simulink model "afe_rst_ctrl"  (R2026b)
settings: Solver=ode23t  StopTime=param.sim.simlength  FixedStep=tc  MaxStep=param.glb_time.tc  RelTol=1e-4
values from neighbouring files (symbols this model uses):
  param = add_template_extras(param, options)    [init_model.m]
undefined symbols (not defined in the file or in its folder): magnitude
libraries: fl_lib x181, nesl_utility x97, igbt_simple_2th_lib x6, afe_uvw_ctrl x5, discrete_time_low_pass_filter x2, threephase_inductor_lib x1, dclink_for_two_levels x1, three_phase_pwm_modulator x1, three_phase_inverter_ideal_switch_based_model x1, three_phase_inverter_mosfet_based_with_thermal_model x1, ee_lib x1, three_phase_voltage_with_frt_emulator_mfcn x1
(part 3 of 6)

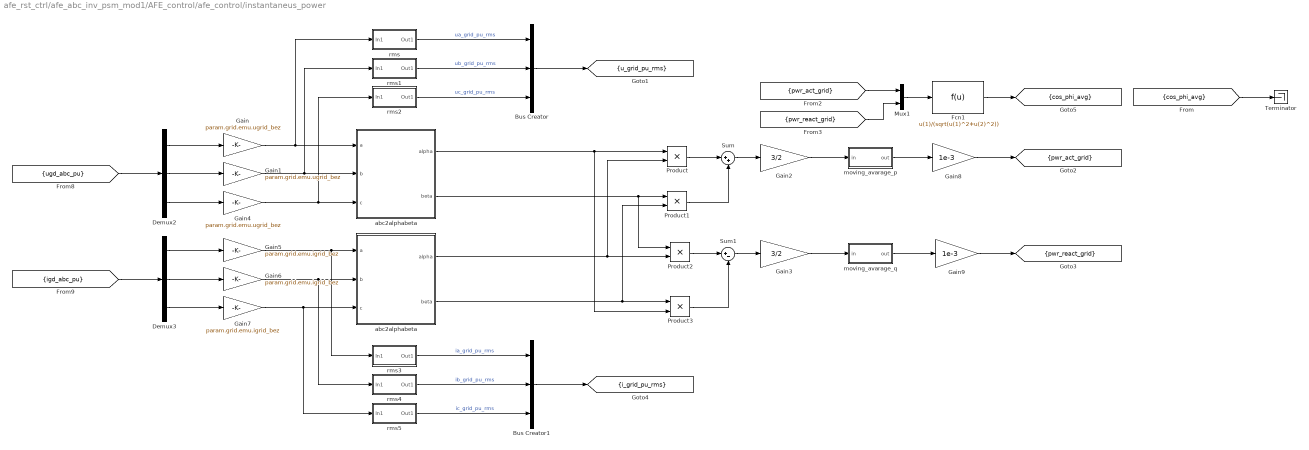
== system afe_rst_ctrl/afe_abc_inv_psm_mod1/AFE_control/afe_control/instantaneus_power ==
  Bus Creator : BusCreator  Inputs=3
  Bus Creator1 : BusCreator  Inputs=3
  Demux2 : Demux  Outputs=3
  Demux3 : Demux  Outputs=3
  Fcn1 : Fcn  Expr=u(1)/(sqrt(u(1)^2+u(2)^2))
  Gain : Gain  Gain=param.grid.emu.ugrid_bez
  Gain1 : Gain  Gain=param.grid.emu.ugrid_bez
  Gain2 : Gain  Gain=3/2
  Gain3 : Gain  Gain=3/2
  Gain4 : Gain  Gain=param.grid.emu.ugrid_bez
  Gain5 : Gain  Gain=param.grid.emu.igrid_bez
  Gain6 : Gain  Gain=param.grid.emu.igrid_bez
  Gain7 : Gain  Gain=param.grid.emu.igrid_bez
  Gain8 : Gain  Gain=1e-3
  Gain9 : Gain  Gain=1e-3
  Mux1 : Mux  Inputs=2
  Product{,1..3} (4 alike) : Product  RndMeth=Zero
  Sum : Sum  Inputs=|++
  Sum1 : Sum  Inputs=|+-
  Terminator : Terminator
  abc2alphabeta : Subsystem
  "abc2alphabeta " : Subsystem
  moving_avarage_p : Subsystem
  moving_avarage_q : Subsystem
  rms : Subsystem
  rms1 : Subsystem
  rms2 : Subsystem
  rms3 : Subsystem
  rms4 : Subsystem
  rms5 : Subsystem
  tag scope: cos_phi_avg=scoped, i_grid_pu_rms=scoped, pwr_act_grid=scoped, pwr_react_grid=scoped, u_grid_pu_rms=scoped
  wires:
  abc2alphabeta/2("beta ") -> Product1/1, Product2/1
  "abc2alphabeta "/2("beta ") -> Product1/2, Product3/1
  abc2alphabeta/1("alpha ") -> Product3/2, Product/1
  "abc2alphabeta "/1("alpha ") -> Product2/2, Product/2
  Product/1 -> Sum/1
  Product1/1 -> Sum/2
  Product2/1 -> Sum1/1
  Product3/1 -> Sum1/2
  Sum1/1 -> Gain3/1
  Sum/1 -> Gain2/1
  Gain2/1 -> moving_avarage_p/1(in)
  Gain3/1 -> moving_avarage_q/1(in)
  [pwr_react_grid] -> Mux1/2
  Mux1/1 -> Fcn1/1
  Fcn1/1 -> [cos_phi_avg]
  [pwr_act_grid] -> Mux1/1
  rms/1(Out1) -> Bus Creator/1  "ua_grid_pu_rms"
  rms2/1(Out1) -> Bus Creator/3  "uc_grid_pu_rms"
  rms1/1(Out1) -> Bus Creator/2  "ub_grid_pu_rms"
  moving_avarage_p/1(out) -> Gain8/1
  moving_avarage_q/1(out) -> Gain9/1
  Demux2/1 -> Gain/1
  Demux2/2 -> Gain1/1
  Demux2/3 -> Gain4/1
  Demux3/1 -> Gain5/1
  Demux3/2 -> Gain6/1
  Demux3/3 -> Gain7/1
  Gain/1 -> rms/1(In1), abc2alphabeta/1(a)
  Gain1/1 -> rms1/1(In1), abc2alphabeta/2(b)
  Gain4/1 -> rms2/1(In1), abc2alphabeta/3(c)
  Gain5/1 -> rms3/1(In1), "abc2alphabeta "/1(a)
  Gain6/1 -> rms4/1(In1), "abc2alphabeta "/2(b)
  Gain7/1 -> rms5/1(In1), "abc2alphabeta "/3(c)
  Gain8/1 -> [pwr_act_grid]
  Gain9/1 -> [pwr_react_grid]
  [ugd_abc_pu] -> Demux2/1
  [igd_abc_pu] -> Demux3/1
  Bus Creator/1 -> [u_grid_pu_rms]
  rms4/1(Out1) -> Bus Creator1/2  "ib_grid_pu_rms"
  rms3/1(Out1) -> Bus Creator1/1  "ia_grid_pu_rms"
  rms5/1(Out1) -> Bus Creator1/3  "ic_grid_pu_rms"
  Bus Creator1/1 -> [i_grid_pu_rms]
  [cos_phi_avg] -> Terminator/1

== system afe_rst_ctrl/afe_abc_inv_psm_mod1/AFE_control/afe_control/interesting scopes ==
  current_sequences_mod1 : Scope  NumInputPorts=4
      settings: ActiveDisplayYMinimum=-0.97178065031766891  ActiveDisplayYMaximum=1.9392475411295891  DataLoggingVariableName=ScopeData2
  i_grid_seq_ref : Scope
      settings: ActiveDisplayYMinimum=-1.1499999999999995  ActiveDisplayYMaximum=0.34999999999999981
  voltage_sequences_mod1 : Scope  NumInputPorts=4
      settings: ActiveDisplayYMinimum=-1.2405151816982258  ActiveDisplayYMaximum=1.2605257614333911
  wires:
  [v_grid_neg_eta_avg] -> voltage_sequences_mod1/4  "u_grid_neg_eta"
  [i_grid_neg_xi_avg] -> current_sequences_mod1/3  "i_grid_neg_xi"
  [v_grid_pos_eta_avg] -> voltage_sequences_mod1/2  "u_grid_pos_eta"
  [v_grid_neg_xi_avg] -> voltage_sequences_mod1/3  "u_grid_neg_xi"
  [i_grid_pos_xi_avg] -> current_sequences_mod1/1  "i_grid_pos_xi"
  [i_grid_neg_eta_avg] -> current_sequences_mod1/4  "i_grid_neg_eta"
  [v_grid_pos_xi_avg] -> voltage_sequences_mod1/1  "u_grid_pos_xi"
  [i_grid_pos_eta_avg] -> current_sequences_mod1/2  "i_grid_pos_eta"
  [i_grid_seq_ref] -> i_grid_seq_ref/1  "i_grid_seq_ref"

== system afe_rst_ctrl/afe_abc_inv_psm_mod1/AFE_control/afe_control/is afe quantizzation and one step delay ==
  is_abc_pu : Inport
  Demux : Demux  Outputs=3
  Mux : Mux  Inputs=3
  is afe quantizzation and one step delay : Subsystem
  isd_abc_pu : Outport
  wires:
  is afe quantizzation and one step delay/2(isd_v_pu) -> Mux/2
  is_abc_pu/1 -> Demux/1
  is afe quantizzation and one step delay/3(isd_w_pu) -> Mux/3
  is afe quantizzation and one step delay/1(isd_u_pu) -> Mux/1
  Demux/1 -> is afe quantizzation and one step delay/1(is_u_pu)
  Mux/1 -> isd_abc_pu/1
  Demux/3 -> is afe quantizzation and one step delay/3(is_w_pu)
  Demux/2 -> is afe quantizzation and one step delay/2(is_v_pu)

== system afe_rst_ctrl/afe_abc_inv_psm_mod1/AFE_control/afe_control/islanding_mode_detector ==
  gamma : Inport
  alpha : Inport  Port=2
  beta : Inport  Port=3
  Constant : Constant
  Mux : Mux  Inputs=2
  island_detection : Scope  NumInputPorts=3
      settings: ActiveDisplayYMinimum=-13.028939727220205  ActiveDisplayYMaximum=117.26045754498188  DataLoggingVariableName=ScopeData10
  islanding_detector : afe_uvw_ctrl/islanding_detector  p=param.afe.uvw
  wires:
  Mux/1 -> islanding_detector/1
  alpha/1 -> Mux/1  "u_grid_alpha"
  beta/1 -> Mux/2  "u_grid_beta"
  gamma/1 -> islanding_detector/2  "gamma_grid"
  [omega_grid_pll_pu] -> islanding_detector/3
  Constant/1 -> islanding_detector/4
  islanding_detector/1 -> island_detection/1
  islanding_detector/2 -> island_detection/2
  islanding_detector/3 -> island_detection/3

== system afe_rst_ctrl/afe_abc_inv_psm_mod1/AFE_control/afe_control/phase_compensation_1 ==
  local_time : Inport
  master_time : Inport  Port=2
  Zero-Order Hold : ZeroOrderHold  SampleTime=-1
  Zero-Order Hold1 : ZeroOrderHold  SampleTime=-1
  alignment_eval_afe1 : Subsystem
  y : Outport
  wires:
  local_time/1 -> Zero-Order Hold/1
  master_time/1 -> Zero-Order Hold1/1
  alignment_eval_afe1/1(dp) -> y/1
  Zero-Order Hold/1 -> alignment_eval_afe1/1(local_time)
  Zero-Order Hold1/1 -> alignment_eval_afe1/2(master_time)

== system afe_rst_ctrl/afe_abc_inv_psm_mod1/AFE_control/afe_control/space_vector ==
  uab_out : Inport
  Bus Creator : BusCreator  Inputs=3
  Bus Selector : BusSelector  OutputSignals=da,db,dc
  C Caller : CCaller  FunctionName=sv_pwm_cm_process_simulink  PortSpecificationStruct="%)30     .    B H   8    (     @         %    \"     8    !     0         %  0 \"0    $    _    07)G3F%M90  4&]R=$YA;64 4V-O<&4     26YD97@     5'EP90      4VEZ90      27-';&]B86P   X    P    !@    @    $          4    (     0    ,    !         !   P!O=70 #@   #     &    \"     0         !0    @    !     P    $         $  # &]U=  .    .     8    (    !          %    \"     $    &     0         0   ...(+3252 chars)"
  Constant : Constant  Value=param.glb_time.ts_afe
  Constant1 : Constant
  Data Type Conversion1 : DataTypeConversion  OutDataTypeStr=double  SaturateOnIntegerOverflow=off  RndMeth=Floor
  Data Type Conversion{4,15..16,18} (4 alike) : DataTypeConversion  OutDataTypeStr=single  SaturateOnIntegerOverflow=off  RndMeth=Floor
  Data Type Conversion17 : DataTypeConversion  OutDataTypeStr=uint32  SaturateOnIntegerOverflow=off  RndMeth=Floor
  Data Type Conversion2 : DataTypeConversion  OutDataTypeStr=double  SaturateOnIntegerOverflow=off  RndMeth=Floor
  Data Type Conversion3 : DataTypeConversion  OutDataTypeStr=double  SaturateOnIntegerOverflow=off  RndMeth=Floor
  Demux : Demux  Outputs=3
  Gain1 : Gain  Gain=sqrt(3)/2
  Gain2 : Gain  Gain=sqrt(3)/2
  Gain3 : Gain  Gain=param.afe.ref.u_cm_comp_mod1
  duvw : Outport
  wires:
  Data Type Conversion15/1 -> C Caller/2
  Bus Selector/2 -> Data Type Conversion2/1  "<db>"
  Data Type Conversion18/1 -> C Caller/1
  C Caller/1 -> Bus Selector/1
  Bus Creator/1 -> duvw/1
  Data Type Conversion1/1 -> Bus Creator/1  "du(k)"
  Demux/2 -> Gain2/1
  Bus Selector/3 -> Data Type Conversion3/1  "<dc>"
  Demux/1 -> Gain1/1
  Data Type Conversion2/1 -> Bus Creator/2  "dv(k)"
  Gain2/1 -> Data Type Conversion15/1
  Bus Selector/1 -> Data Type Conversion1/1  "<da>"
  Gain1/1 -> Data Type Conversion18/1
  Data Type Conversion3/1 -> Bus Creator/3  "dw(k)"
  Constant/1 -> Data Type Conversion16/1
  uab_out/1 -> Demux/1
  Constant1/1 -> Data Type Conversion17/1
  Data Type Conversion16/1 -> C Caller/4
  Data Type Conversion17/1 -> C Caller/5
  Demux/3 -> Gain3/1
  Gain3/1 -> Data Type Conversion4/1
  Data Type Conversion4/1 -> C Caller/3

== system afe_rst_ctrl/afe_abc_inv_psm_mod1/AFE_control/afe_control/udc_acquisition ==
  udc_pu : Inport
  Quantizer : Quantizer  QuantizationInterval=param.meas.adc_quantization
  Unit Delay : UnitDelay  SampleTime=-1
  Zero-Order Hold : ZeroOrderHold  SampleTime=-1
  udcd_pu : Outport
  wires:
  Quantizer/1 -> Unit Delay/1
  udc_pu/1 -> Zero-Order Hold/1
  Unit Delay/1 -> udcd_pu/1
  Zero-Order Hold/1 -> Quantizer/1

== system afe_rst_ctrl/afe_abc_inv_psm_mod1/AFE_control/afe_control/udc_ctrl ==
  udc_pu : Inport
  1/Ti : Gain  Gain=param.afe.ctrl.kp_udc_ctrl  SaturateOnIntegerOverflow=on  OutDataTypeStr=Inherit: Same as input  ParamDataTypeStr=Inherit: Same as input
  Constant : Constant  Value=0
  Gain : Gain  Gain=-1
  Saturation : Saturate  UpperLimit=param.afe.ctrl.ixi_pos_ref_lim  LowerLimit=-param.afe.ctrl.ixi_pos_ref_lim
  Sum1 : Sum  Inputs=+++  SaturateOnIntegerOverflow=on
  Sum2 : Sum  Inputs=-+  SaturateOnIntegerOverflow=on
  Sum3 : Sum  Inputs=-+  SaturateOnIntegerOverflow=on
  Switch : Switch  Criteria=u2 > Threshold  SaturateOnIntegerOverflow=off  InputSameDT=off
  To Workspace1 : ToWorkspace  VariableName=udc_pu_sim_mod1  SampleTime=-1
      settings: MaxDataPoints=param.glb_time.Ns_afe
  To Workspace3 : ToWorkspace  VariableName=udc_pu_ref_sim_mod1  SampleTime=-1
      settings: MaxDataPoints=param.glb_time.Ns_afe
  Unit Delay4 : UnitDelay  SampleTime=-1
  discrete-time-low-pass-filter1 : discrete_time_low_pass_filter/discrete-time-low-pass-filter  tau=20e-3  ts=param.glb_time.ts_afe
  kp : Gain  Gain=param.afe.ctrl.ki_udc_ctrl*param.glb_time.ts_afe  SaturateOnIntegerOverflow=on  OutDataTypeStr=Inherit: Same as input  ParamDataTypeStr=Inherit: Same as input
  udc_norm_ref : Step  Time=1e-3  FinalValue=param.afe.ctrl.udc_norm_ref
  udc_tracking : Scope  NumInputPorts=3
      settings: ActiveDisplayYMinimum=-2.0004150390624997  ActiveDisplayYMaximum=1.5037353515624998  DataLoggingVariableName=ScopeData8
  i_xi_ref : Outport
  wires:
  1/Ti/1 -> Sum1/1, Sum3/1
  kp/1 -> Sum1/2
  Sum3/1 -> Unit Delay4/1
  Unit Delay4/1 -> Sum1/3
  udc_norm_ref/1 -> discrete-time-low-pass-filter1/1
  udc_pu/1 -> Sum2/1, To Workspace1/1, udc_tracking/2  "udc_pu"
  Sum2/1 -> kp/1, 1/Ti/1
  Sum1/1 -> Saturation/1
  [pwr_lim_enable] -> Switch/2
  Saturation/1 -> Switch/3
  Switch/1 -> Sum3/2, Gain/1
  Constant/1 -> Switch/1
  Gain/1 -> udc_tracking/3, i_xi_ref/1  "i_xi_ref"
  discrete-time-low-pass-filter1/1 -> To Workspace3/1, udc_tracking/1, Sum2/2  "udc_pu_ref"

== system afe_rst_ctrl/afe_abc_inv_psm_mod1/AFE_control/afe_control/ug afe quantizzation and one step delay ==
  ug_abc_pu : Inport
  Demux : Demux  Outputs=3
  Mux : Mux  Inputs=3
  ug afe quantizzation and one step delay : Subsystem
  ugd_abc_pu : Outport
  wires:
  ug afe quantizzation and one step delay/2(ugd_v_pu) -> Mux/2
  Demux/2 -> ug afe quantizzation and one step delay/2(ug_v_pu)
  Demux/3 -> ug afe quantizzation and one step delay/3(ug_w_pu)
  ug afe quantizzation and one step delay/1(ugd_u_pu) -> Mux/1
  Demux/1 -> ug afe quantizzation and one step delay/1(ug_u_pu)
  ug_abc_pu/1 -> Demux/1
  ug afe quantizzation and one step delay/3(ugd_w_pu) -> Mux/3
  Mux/1 -> ugd_abc_pu/1

== system afe_rst_ctrl/afe_abc_inv_psm_mod1/afe/sv_pwm/modulator1 ==
  u : Inport
  v : Inport  Port=2
  w : Inport  Port=3
  phase : Inport  Port=4
  Bus Creator : BusCreator  Inputs=3
  Three phase two level PWM generator with global TRGO : three_phase_pwm_modulator/Three phase two level PWM generator with global TRGO  f=param.glb_time.fPWM_AFE  m_up=0.98  m_low=0.02  dead_time=param.glb_time.dead_time_AFE  pos_cmd_gate=15  neg_cmd_gate=-10  polarity=1  tc=param.glb_time.tc  double_sampling=1
      link override gate commands/Bus Selector: OutputSignals=du(t)
      link override gate commands/Bus Selector1: OutputSignals=dv(t)
      link override gate commands/Bus Selector2: OutputSignals=dw(t)
  gate_cmds : Outport
  tag scope: TRGO_afe_module_1=global
  wires:
  [time_afe_module_1] -> Three phase two level PWM generator with global TRGO/1
  Bus Creator/1 -> Three phase two level PWM generator with global TRGO/3
  Three phase two level PWM generator with global TRGO/1 -> [TRGO_afe_module_1]
  u/1 -> Bus Creator/1
  v/1 -> Bus Creator/2
  w/1 -> Bus Creator/3
  phase/1 -> Three phase two level PWM generator with global TRGO/2
  Three phase two level PWM generator with global TRGO/2 -> gate_cmds/1

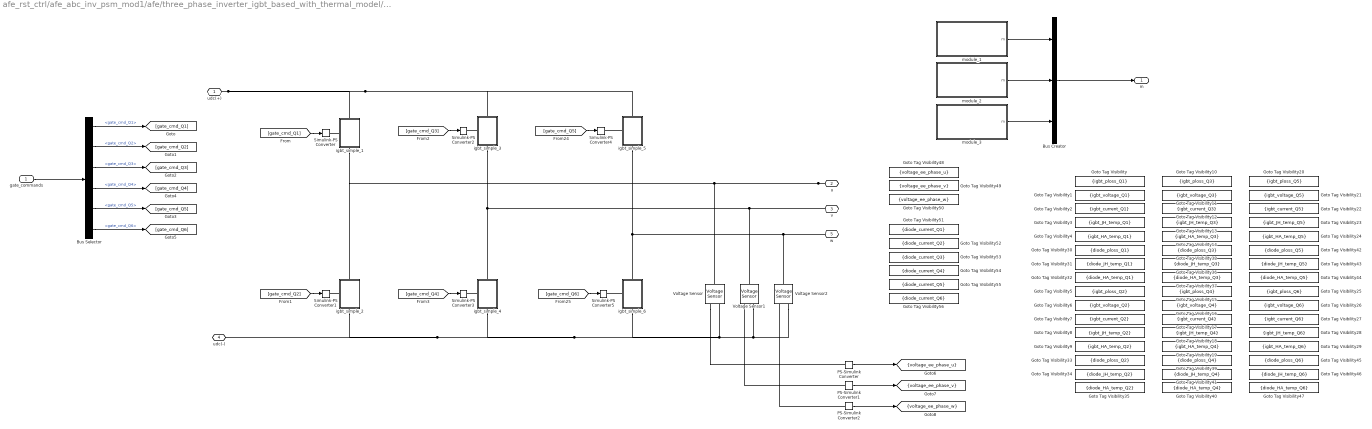
== system afe_rst_ctrl/afe_abc_inv_psm_mod1/afe/three_phase_inverter_igbt_based_with_thermal_model/three_phase_inverter_with_igbt_simple_2th ==
  gate_commands : Inport
  Bus Creator : BusCreator  Inputs=3
  Bus Selector : BusSelector  OutputSignals=gate_cmd_Q1,gate_cmd_Q2,gate_cmd_Q3,gate_cmd_Q4,gate_cmd_Q5,gate_cmd_Q6
  Goto Tag Visibility : GotoTagVisibility  GotoTag=igbt_ploss_Q1
  Goto Tag Visibility1 : GotoTagVisibility  GotoTag=igbt_voltage_Q1
  Goto Tag Visibility10 : GotoTagVisibility  GotoTag=igbt_ploss_Q3
  Goto Tag Visibility11 : GotoTagVisibility  GotoTag=igbt_voltage_Q3
  Goto Tag Visibility12 : GotoTagVisibility  GotoTag=igbt_current_Q3
  Goto Tag Visibility13 : GotoTagVisibility  GotoTag=igbt_JH_temp_Q3
  Goto Tag Visibility14 : GotoTagVisibility  GotoTag=igbt_HA_temp_Q3
  Goto Tag Visibility15 : GotoTagVisibility  GotoTag=igbt_ploss_Q4
  Goto Tag Visibility16 : GotoTagVisibility  GotoTag=igbt_voltage_Q4
  Goto Tag Visibility17 : GotoTagVisibility  GotoTag=igbt_current_Q4
  Goto Tag Visibility18 : GotoTagVisibility  GotoTag=igbt_JH_temp_Q4
  Goto Tag Visibility19 : GotoTagVisibility  GotoTag=igbt_HA_temp_Q4
  Goto Tag Visibility2 : GotoTagVisibility  GotoTag=igbt_current_Q1
  Goto Tag Visibility20 : GotoTagVisibility  GotoTag=igbt_ploss_Q5
  Goto Tag Visibility21 : GotoTagVisibility  GotoTag=igbt_voltage_Q5
  Goto Tag Visibility22 : GotoTagVisibility  GotoTag=igbt_current_Q5
  Goto Tag Visibility23 : GotoTagVisibility  GotoTag=igbt_JH_temp_Q5
  Goto Tag Visibility24 : GotoTagVisibility  GotoTag=igbt_HA_temp_Q5
  Goto Tag Visibility25 : GotoTagVisibility  GotoTag=igbt_ploss_Q6
  Goto Tag Visibility26 : GotoTagVisibility  GotoTag=igbt_voltage_Q6
  Goto Tag Visibility27 : GotoTagVisibility  GotoTag=igbt_current_Q6
  Goto Tag Visibility28 : GotoTagVisibility  GotoTag=igbt_JH_temp_Q6
  Goto Tag Visibility29 : GotoTagVisibility  GotoTag=igbt_HA_temp_Q6
  Goto Tag Visibility3 : GotoTagVisibility  GotoTag=igbt_JH_temp_Q1
  Goto Tag Visibility30 : GotoTagVisibility  GotoTag=diode_ploss_Q1
  Goto Tag Visibility31 : GotoTagVisibility  GotoTag=diode_JH_temp_Q1
  Goto Tag Visibility32 : GotoTagVisibility  GotoTag=diode_HA_temp_Q1
  Goto Tag Visibility33 : GotoTagVisibility  GotoTag=diode_ploss_Q2
  Goto Tag Visibility34 : GotoTagVisibility  GotoTag=diode_JH_temp_Q2
  Goto Tag Visibility35 : GotoTagVisibility  GotoTag=diode_HA_temp_Q2
  Goto Tag Visibility36 : GotoTagVisibility  GotoTag=diode_JH_temp_Q3
  Goto Tag Visibility37 : GotoTagVisibility  GotoTag=diode_HA_temp_Q3
  Goto Tag Visibility38 : GotoTagVisibility  GotoTag=diode_ploss_Q3
  Goto Tag Visibility39 : GotoTagVisibility  GotoTag=diode_ploss_Q4
  Goto Tag Visibility4 : GotoTagVisibility  GotoTag=igbt_HA_temp_Q1
  Goto Tag Visibility40 : GotoTagVisibility  GotoTag=diode_HA_temp_Q4
  Goto Tag Visibility41 : GotoTagVisibility  GotoTag=diode_JH_temp_Q4
  Goto Tag Visibility42 : GotoTagVisibility  GotoTag=diode_ploss_Q5
  Goto Tag Visibility43 : GotoTagVisibility  GotoTag=diode_JH_temp_Q5
  Goto Tag Visibility44 : GotoTagVisibility  GotoTag=diode_HA_temp_Q5
  Goto Tag Visibility45 : GotoTagVisibility  GotoTag=diode_ploss_Q6
  Goto Tag Visibility46 : GotoTagVisibility  GotoTag=diode_JH_temp_Q6
  Goto Tag Visibility47 : GotoTagVisibility  GotoTag=diode_HA_temp_Q6
  Goto Tag Visibility48 : GotoTagVisibility  GotoTag=voltage_ee_phase_u
  Goto Tag Visibility49 : GotoTagVisibility  GotoTag=voltage_ee_phase_v
  Goto Tag Visibility5 : GotoTagVisibility  GotoTag=igbt_ploss_Q2
  Goto Tag Visibility50 : GotoTagVisibility  GotoTag=voltage_ee_phase_w
  Goto Tag Visibility51 : GotoTagVisibility  GotoTag=diode_current_Q1
  Goto Tag Visibility52 : GotoTagVisibility  GotoTag=diode_current_Q2
  Goto Tag Visibility53 : GotoTagVisibility  GotoTag=diode_current_Q3
  Goto Tag Visibility54 : GotoTagVisibility  GotoTag=diode_current_Q4
  Goto Tag Visibility55 : GotoTagVisibility  GotoTag=diode_current_Q5
  Goto Tag Visibility56 : GotoTagVisibility  GotoTag=diode_current_Q6
  Goto Tag Visibility6 : GotoTagVisibility  GotoTag=igbt_voltage_Q2
  Goto Tag Visibility7 : GotoTagVisibility  GotoTag=igbt_current_Q2
  Goto Tag Visibility8 : GotoTagVisibility  GotoTag=igbt_JH_temp_Q2
  Goto Tag Visibility9 : GotoTagVisibility  GotoTag=igbt_HA_temp_Q2
  PS-Simulink Converter : nesl_utility/PS-Simulink Converter  PhysicalDomain=network_engine_domain  SubClassName=ps_output  LeftPortType=input  RightPortType=output  PseudoPeriodic=off  Frequencies=[]  VectorFormat=1-D array  Unit=V  AffineConversion=off
  PS-Simulink Converter1 : nesl_utility/PS-Simulink Converter  PhysicalDomain=network_engine_domain  SubClassName=ps_output  LeftPortType=input  RightPortType=output  PseudoPeriodic=off  Frequencies=[]  VectorFormat=1-D array  Unit=V  AffineConversion=off
  PS-Simulink Converter2 : nesl_utility/PS-Simulink Converter  PhysicalDomain=network_engine_domain  SubClassName=ps_output  LeftPortType=input  RightPortType=output  PseudoPeriodic=off  Frequencies=[]  VectorFormat=1-D array  Unit=V  AffineConversion=off
  Simulink-PS Converter{,1..5} (6 alike) : nesl_utility/Simulink-PS Converter  PhysicalDomain=network_engine_domain  SubClassName=ps_input  LeftPortType=input  RightPortType=output  PseudoPeriodic=off  Frequencies=[]  NoiseDistribution=none  NoiseParameters=[]  Unit=V  AffineConversion=off  FilteringAndDerivatives=provide  SimscapeFilterOrder=1  InputFilterTimeConstant=0.001  UdotUserProvided=0
  Voltage Sensor : fl_lib/Electrical/Electrical Sensors/Voltage Sensor
  Voltage Sensor1 : fl_lib/Electrical/Electrical Sensors/Voltage Sensor
  Voltage Sensor2 : fl_lib/Electrical/Electrical Sensors/Voltage Sensor
  igbt_simple_1 : Subsystem
      settings: PortSchema="{\"entries\":[{\"content\":{\"sides\":[{\"content\":{\"connectorIds\":[\"LConn1\"]},\"type\":\"ConnectorPlacement.EquallySpacedRectSide\",\"uuid\":\"9277da8d-d460-43e6-8478-dd662f15d226\"},{\"content\":{\"connectorIds\":[],\"side\":\"RIGHT\"},\"type\":\"ConnectorPlacement.EquallySpacedRectSide\",\"uuid\":\"a7ece396-f1d9-4f4f-a05b-db1fc65d6e1d\"},{\"content\":{\"connectorIds\":[\"LConn2\"],\"side\":\"TOP\"},\"type\":\"ConnectorPlacement.EquallySpacedRectSide\",\"uuid\":\"fdd70777-e9cf-4317-afb6-cae87f75d5b0\"},{\"content\":{\"connectorIds\":[\"RConn1\"],\"side\":\"BOTTOM\"},\"type\":\"ConnectorPlacement.EquallySpacedRectSide\",\"uuid\":\"2353ed68-b1a1-4775-9ca9-31e268d5443b\"}]},\"type\":\"ConnectorPlacement.EquallySpacedConnector\",\"uuid\":\"d5479f4c-4e65-4791-adcb-73df11f88590\"}],\"packageUris\":[\"http://schema.mathworks.com/mf0/Connector/R2020b\"],\"version\":\"1.0\"}"
  igbt_simple_2 : Subsystem
      settings: PortSchema="{\"entries\":[{\"content\":{\"sides\":[{\"content\":{\"connectorIds\":[\"LConn1\"]},\"type\":\"ConnectorPlacement.EquallySpacedRectSide\",\"uuid\":\"9277da8d-d460-43e6-8478-dd662f15d226\"},{\"content\":{\"connectorIds\":[],\"side\":\"RIGHT\"},\"type\":\"ConnectorPlacement.EquallySpacedRectSide\",\"uuid\":\"a7ece396-f1d9-4f4f-a05b-db1fc65d6e1d\"},{\"content\":{\"connectorIds\":[\"LConn2\"],\"side\":\"TOP\"},\"type\":\"ConnectorPlacement.EquallySpacedRectSide\",\"uuid\":\"fdd70777-e9cf-4317-afb6-cae87f75d5b0\"},{\"content\":{\"connectorIds\":[\"RConn1\"],\"side\":\"BOTTOM\"},\"type\":\"ConnectorPlacement.EquallySpacedRectSide\",\"uuid\":\"2353ed68-b1a1-4775-9ca9-31e268d5443b\"}]},\"type\":\"ConnectorPlacement.EquallySpacedConnector\",\"uuid\":\"d5479f4c-4e65-4791-adcb-73df11f88590\"}],\"packageUris\":[\"http://schema.mathworks.com/mf0/Connector/R2020b\"],\"version\":\"1.0\"}"
  igbt_simple_3 : Subsystem
      settings: PortSchema="{\"entries\":[{\"content\":{\"sides\":[{\"content\":{\"connectorIds\":[\"LConn1\"]},\"type\":\"ConnectorPlacement.EquallySpacedRectSide\",\"uuid\":\"9277da8d-d460-43e6-8478-dd662f15d226\"},{\"content\":{\"connectorIds\":[],\"side\":\"RIGHT\"},\"type\":\"ConnectorPlacement.EquallySpacedRectSide\",\"uuid\":\"a7ece396-f1d9-4f4f-a05b-db1fc65d6e1d\"},{\"content\":{\"connectorIds\":[\"LConn2\"],\"side\":\"TOP\"},\"type\":\"ConnectorPlacement.EquallySpacedRectSide\",\"uuid\":\"fdd70777-e9cf-4317-afb6-cae87f75d5b0\"},{\"content\":{\"connectorIds\":[\"RConn1\"],\"side\":\"BOTTOM\"},\"type\":\"ConnectorPlacement.EquallySpacedRectSide\",\"uuid\":\"2353ed68-b1a1-4775-9ca9-31e268d5443b\"}]},\"type\":\"ConnectorPlacement.EquallySpacedConnector\",\"uuid\":\"d5479f4c-4e65-4791-adcb-73df11f88590\"}],\"packageUris\":[\"http://schema.mathworks.com/mf0/Connector/R2020b\"],\"version\":\"1.0\"}"
  igbt_simple_4 : Subsystem
      settings: PortSchema="{\"entries\":[{\"content\":{\"sides\":[{\"content\":{\"connectorIds\":[\"LConn1\"]},\"type\":\"ConnectorPlacement.EquallySpacedRectSide\",\"uuid\":\"9277da8d-d460-43e6-8478-dd662f15d226\"},{\"content\":{\"connectorIds\":[],\"side\":\"RIGHT\"},\"type\":\"ConnectorPlacement.EquallySpacedRectSide\",\"uuid\":\"a7ece396-f1d9-4f4f-a05b-db1fc65d6e1d\"},{\"content\":{\"connectorIds\":[\"LConn2\"],\"side\":\"TOP\"},\"type\":\"ConnectorPlacement.EquallySpacedRectSide\",\"uuid\":\"fdd70777-e9cf-4317-afb6-cae87f75d5b0\"},{\"content\":{\"connectorIds\":[\"RConn1\"],\"side\":\"BOTTOM\"},\"type\":\"ConnectorPlacement.EquallySpacedRectSide\",\"uuid\":\"2353ed68-b1a1-4775-9ca9-31e268d5443b\"}]},\"type\":\"ConnectorPlacement.EquallySpacedConnector\",\"uuid\":\"d5479f4c-4e65-4791-adcb-73df11f88590\"}],\"packageUris\":[\"http://schema.mathworks.com/mf0/Connector/R2020b\"],\"version\":\"1.0\"}"
  igbt_simple_5 : Subsystem
      settings: PortSchema="{\"entries\":[{\"content\":{\"sides\":[{\"content\":{\"connectorIds\":[\"LConn1\"]},\"type\":\"ConnectorPlacement.EquallySpacedRectSide\",\"uuid\":\"9277da8d-d460-43e6-8478-dd662f15d226\"},{\"content\":{\"connectorIds\":[],\"side\":\"RIGHT\"},\"type\":\"ConnectorPlacement.EquallySpacedRectSide\",\"uuid\":\"a7ece396-f1d9-4f4f-a05b-db1fc65d6e1d\"},{\"content\":{\"connectorIds\":[\"LConn2\"],\"side\":\"TOP\"},\"type\":\"ConnectorPlacement.EquallySpacedRectSide\",\"uuid\":\"fdd70777-e9cf-4317-afb6-cae87f75d5b0\"},{\"content\":{\"connectorIds\":[\"RConn1\"],\"side\":\"BOTTOM\"},\"type\":\"ConnectorPlacement.EquallySpacedRectSide\",\"uuid\":\"2353ed68-b1a1-4775-9ca9-31e268d5443b\"}]},\"type\":\"ConnectorPlacement.EquallySpacedConnector\",\"uuid\":\"d5479f4c-4e65-4791-adcb-73df11f88590\"}],\"packageUris\":[\"http://schema.mathworks.com/mf0/Connector/R2020b\"],\"version\":\"1.0\"}"
  igbt_simple_6 : Subsystem
      settings: PortSchema="{\"entries\":[{\"content\":{\"sides\":[{\"content\":{\"connectorIds\":[\"LConn1\"]},\"type\":\"ConnectorPlacement.EquallySpacedRectSide\",\"uuid\":\"9277da8d-d460-43e6-8478-dd662f15d226\"},{\"content\":{\"connectorIds\":[],\"side\":\"RIGHT\"},\"type\":\"ConnectorPlacement.EquallySpacedRectSide\",\"uuid\":\"a7ece396-f1d9-4f4f-a05b-db1fc65d6e1d\"},{\"content\":{\"connectorIds\":[\"LConn2\"],\"side\":\"TOP\"},\"type\":\"ConnectorPlacement.EquallySpacedRectSide\",\"uuid\":\"fdd70777-e9cf-4317-afb6-cae87f75d5b0\"},{\"content\":{\"connectorIds\":[\"RConn1\"],\"side\":\"BOTTOM\"},\"type\":\"ConnectorPlacement.EquallySpacedRectSide\",\"uuid\":\"2353ed68-b1a1-4775-9ca9-31e268d5443b\"}]},\"type\":\"ConnectorPlacement.EquallySpacedConnector\",\"uuid\":\"d5479f4c-4e65-4791-adcb-73df11f88590\"}],\"packageUris\":[\"http://schema.mathworks.com/mf0/Connector/R2020b\"],\"version\":\"1.0\"}"
  module_1 : Subsystem
  module_2 : Subsystem
  module_3 : Subsystem
  udc(+) : PMIOPort  Side=Left
  u : PMIOPort  Port=2  Side=Right
  v : PMIOPort  Port=3  Side=Right
  udc(-) : PMIOPort  Port=4  Side=Left
  w : PMIOPort  Port=5  Side=Right
  m : Outport
  tag scope: voltage_ee_phase_u=scoped, voltage_ee_phase_v=scoped, voltage_ee_phase_w=scoped
  wires:
  module_3/1(m) -> Bus Creator/3
  module_1/1(m) -> Bus Creator/1
  Bus Creator/1 -> m/1
  module_2/1(m) -> Bus Creator/2
  PS-Simulink Converter2/1 -> [voltage_ee_phase_w]
  PS-Simulink Converter1/1 -> [voltage_ee_phase_v]
  PS-Simulink Converter/1 -> [voltage_ee_phase_u]
  Bus Selector/6 -> [gate_cmd_Q6]  "<gate_cmd_Q6>"
  Bus Selector/5 -> [gate_cmd_Q5]  "<gate_cmd_Q5>"
  [gate_cmd_Q6] -> Simulink-PS Converter5/1
  [gate_cmd_Q5] -> Simulink-PS Converter4/1
  [gate_cmd_Q3] -> Simulink-PS Converter2/1
  Bus Selector/2 -> [gate_cmd_Q2]  "<gate_cmd_Q2>"
  Bus Selector/1 -> [gate_cmd_Q1]  "<gate_cmd_Q1>"
  Bus Selector/3 -> [gate_cmd_Q3]  "<gate_cmd_Q3>"
  [gate_cmd_Q4] -> Simulink-PS Converter3/1
  [gate_cmd_Q2] -> Simulink-PS Converter1/1
  [gate_cmd_Q1] -> Simulink-PS Converter/1
  Bus Selector/4 -> [gate_cmd_Q4]  "<gate_cmd_Q4>"
  gate_commands/1 -> Bus Selector/1
  connections:
  PS-Simulink Converter2/LConn1 -- Voltage Sensor2/RConn1
  PS-Simulink Converter1/LConn1 -- Voltage Sensor1/RConn1
  Voltage Sensor/RConn1 -- PS-Simulink Converter/LConn1
  w/RConn1 -- Voltage Sensor2/LConn1 -- igbt_simple_6/LConn2 -- igbt_simple_5/RConn1
  v/RConn1 -- Voltage Sensor1/LConn1 -- igbt_simple_4/LConn2 -- igbt_simple_3/RConn1
  Voltage Sensor1/RConn2 -- Voltage Sensor2/RConn2 -- Voltage Sensor/RConn2 -- igbt_simple_6/RConn1 -- igbt_simple_4/RConn1 -- igbt_simple_2/RConn1 -- udc(-)/RConn1
  igbt_simple_6/LConn1 -- Simulink-PS Converter5/RConn1
  igbt_simple_5/LConn1 -- Simulink-PS Converter4/RConn1
  igbt_simple_4/LConn1 -- Simulink-PS Converter3/RConn1
  igbt_simple_3/LConn1 -- Simulink-PS Converter2/RConn1
  igbt_simple_2/LConn1 -- Simulink-PS Converter1/RConn1
  igbt_simple_1/LConn1 -- Simulink-PS Converter/RConn1
  udc(+)/RConn1 -- igbt_simple_1/LConn2 -- igbt_simple_5/LConn2 -- igbt_simple_3/LConn2
  u/RConn1 -- Voltage Sensor/LConn1 -- igbt_simple_2/LConn2 -- igbt_simple_1/RConn1

== system afe_rst_ctrl/afe_abc_inv_psm_mod1/AFE_control/afe_control/FRT-VDE4110/positive_reactive_current_reference ==
  Step : Step  Time=param.afe.ref.time_i_react_pos_ref_1  InitialValue=param.afe.ref.i_react_pos_ref_1  FinalValue=param.afe.ref.i_react_pos_ref_2
  Step1 : Step  Time=param.afe.ref.time_i_react_pos_ref_2  FinalValue=param.afe.ref.i_react_pos_ref_3-param.afe.ref.i_react_pos_ref_2
  Sum7 : Sum  Inputs=|++
  i_react_pos_ref : Outport
  wires:
  Sum7/1 -> i_react_pos_ref/1
  Step1/1 -> Sum7/2
  Step/1 -> Sum7/1

== system afe_rst_ctrl/afe_abc_inv_psm_mod1/AFE_control/afe_control/current_ctrl1/current_transformation ==
  is_a_pu : Inport
  is_b_pu : Inport  Port=2
  is_c_pu : Inport  Port=3
  alphabeta2xieta : MATLAB Function  TreatAsAtomicUnit=on
  uvw2alphabeta : MATLAB Function  TreatAsAtomicUnit=on
  tag scope: id_eta_pu=scoped, id_xi_pu=scoped
  wires:
  is_c_pu/1 -> uvw2alphabeta/3(w)
  alphabeta2xieta/2(eta) -> [id_eta_pu]  "ieta_pu"
  alphabeta2xieta/1(xi) -> [id_xi_pu]  "ixi_pu"
  is_b_pu/1 -> uvw2alphabeta/2(v)
  uvw2alphabeta/2(beta) -> alphabeta2xieta/2(beta)  "ibeta_pu"
  uvw2alphabeta/1(alpha) -> alphabeta2xieta/1(alpha)  "ialpha_pu"
  [phase_grid_pll] -> alphabeta2xieta/3(gamma)
  is_a_pu/1 -> uvw2alphabeta/1(u)

== system afe_rst_ctrl/afe_abc_inv_psm_mod1/AFE_control/afe_control/current_ctrl1/inner_current_ctrl ==
  In1 : Inport
  is_abc : Inport  Port=2
  Mux : Mux  Inputs=3
  Selector : Selector  InputPortWidth=3  IndexOptions=Index vector (dialog)  Indices=[1]  OutputSizes=1  RuntimeRangeChecks=off
  Selector1 : Selector  InputPortWidth=3  IndexOptions=Index vector (dialog)  Indices=[1]  OutputSizes=1  RuntimeRangeChecks=off
  Selector2 : Selector  InputPortWidth=3  IndexOptions=Index vector (dialog)  Indices=[2]  OutputSizes=1  RuntimeRangeChecks=off
  Selector3 : Selector  InputPortWidth=3  IndexOptions=Index vector (dialog)  Indices=[2]  OutputSizes=1  RuntimeRangeChecks=off
  Selector4 : Selector  InputPortWidth=3  IndexOptions=Index vector (dialog)  Indices=[3]  OutputSizes=1  RuntimeRangeChecks=off
  Selector5 : Selector  InputPortWidth=3  IndexOptions=Index vector (dialog)  Indices=[3]  OutputSizes=1  RuntimeRangeChecks=off
  isa_ref/isa : Scope  NumInputPorts=2
      settings: ActiveDisplayYMinimum=0.46634443711045703  ActiveDisplayYMaximum=1.1209185909366344
  isb_ref/isb : Scope  NumInputPorts=2
      settings: ActiveDisplayYMinimum=-1.381866613392059  ActiveDisplayYMaximum=1.3822246036957448  DataLoggingVariableName=ScopeData2
  isc_ref/isc : Scope  NumInputPorts=2
      settings: ActiveDisplayYMinimum=-1.9270596811485752  ActiveDisplayYMaximum=1.9769102920110639  DataLoggingVariableName=ScopeData3
  rpi_phase_a : Subsystem
  rpi_phase_b : Subsystem
  rpi_phase_c : Subsystem
  zero_current_ctrl : Subsystem
  uabg : Outport  VectorParamsAs1DForOutWhenUnconnected=off
  tag scope: isa=scoped, isa_ref=scoped, isb=scoped, isb_ref=scoped, isc=scoped, isc_ref=scoped
  wires:
  In1/1 -> Selector4/1, Selector2/1, Selector/1  "isd_abc_pu_ref"
  is_abc/1 -> Selector5/1, Selector3/1, Selector1/1  "isd_abc_pu"
  Selector/1 -> [isa_ref], isa_ref/isa/1, rpi_phase_a/1(In1)  "isa_ref"
  Selector1/1 -> [isa], isa_ref/isa/2, rpi_phase_a/2(In2)  "isa"
  Selector2/1 -> rpi_phase_b/1(In1), [isb_ref], isb_ref/isb/1  "isb_ref"
  Selector3/1 -> rpi_phase_b/2(In2), [isb], isb_ref/isb/2  "isb"
  Selector4/1 -> rpi_phase_c/1(In1), [isc_ref], isc_ref/isc/1  "isc_ref"
  Selector5/1 -> rpi_phase_c/2(In2), [isc], isc_ref/isc/2  "isc"
  rpi_phase_a/1(Out1) -> Mux/1  "da"
  rpi_phase_b/1(Out1) -> Mux/2  "db"
  rpi_phase_c/1(Out1) -> Mux/3  "dc"
  Mux/1 -> zero_current_ctrl/1(d_abc)  "d_abc"
  zero_current_ctrl/1(u_ctrl_out) -> uabg/1

== system afe_rst_ctrl/afe_abc_inv_psm_mod1/AFE_control/afe_control/current_ctrl1/xieta2abc_ref ==
  pos_xi_ref : Inport
  pos_eta : Inport  Port=2
  neg_xi : Inport  Port=3
  neg_eta : Inport  Port=4
  phase : Inport  Port=5
  MATLAB Function2 : MATLAB Function  TreatAsAtomicUnit=on
  Mux : Mux  Inputs=3
  Negative Sequence : MATLAB Function  TreatAsAtomicUnit=on
  Positive Sequence : MATLAB Function  TreatAsAtomicUnit=on
  Sum : Sum  Inputs=|++
  Sum1 : Sum  Inputs=|++
  i_abc_ref : Outport
  wires:
  neg_eta/1 -> Negative Sequence/2(eta)
  MATLAB Function2/1(a) -> Mux/1  "i_a"
  Positive Sequence/2(beta) -> Sum1/1
  Sum/1 -> MATLAB Function2/1(alpha)
  phase/1 -> Negative Sequence/3(phase), Positive Sequence/3(phase)
  MATLAB Function2/3(c) -> Mux/3  "i_c"
  Negative Sequence/1(alpha) -> Sum/2
  Positive Sequence/1(alpha) -> Sum/1
  Negative Sequence/2(beta) -> Sum1/2
  MATLAB Function2/2(b) -> Mux/2  "i_b"
  Sum1/1 -> MATLAB Function2/2(beta)
  neg_xi/1 -> Negative Sequence/1(xi)
  pos_xi_ref/1 -> Positive Sequence/1(xi)
  pos_eta/1 -> Positive Sequence/2(eta)
  Mux/1 -> i_abc_ref/1  "i_abc"

== system afe_rst_ctrl/afe_abc_inv_psm_mod1/AFE_control/afe_control/data_to_worspace_module_1/dq_pll ==
  Bus Creator1 : BusCreator  Inputs=8
  dqPLLs : Outport
  wires:
  [phase_grid_fht_simulink_pll] -> Bus Creator1/5  "phase_grid_fht_simulink_pll"
  [omega_grid_fht_simulink_pll] -> Bus Creator1/6  "omega_grid_fht_simulink_pll"
  [omega_grid_fhtsr_dqpll] -> Bus Creator1/8  "omega_grid_fhtsr_dqpll"
  [phase_grid_fhtsr_dqpll] -> Bus Creator1/7  "phase_grid_fhtsr_dqpll"
  [omega_grid_dqpll_ccaller] -> Bus Creator1/4  "omega_grid_dqpll_ccaller"
  [phase_grid_dqpll_ccaller] -> Bus Creator1/3  "phase_grid_dqpll_ccaller"
  [omega_grid_pu_dqpll] -> Bus Creator1/2  "omega_grid_pu_dqpll"
  [phase_grid_dqpll] -> Bus Creator1/1  "phase_grid_dqpll"
  Bus Creator1/1 -> dqPLLs/1

== system afe_rst_ctrl/afe_abc_inv_psm_mod1/AFE_control/afe_control/data_to_worspace_module_1/inner_current_tracking ==
  Bus Creator1 : BusCreator  Inputs=11
  m_inner_current_tracking : Outport
  wires:
  [iz_pu] -> Bus Creator1/10  "iz_pu"
  [id_eta_pu] -> Bus Creator1/2  "i_eta_pu"
  [isc] -> Bus Creator1/8  "isc_pu"
  [isa_ref] -> Bus Creator1/3  "isa_pu_ref"
  [isa] -> Bus Creator1/4  "isa_pu"
  [id_xi_pu] -> Bus Creator1/1  "i_xi_pu"
  [iz_pu_ref] -> Bus Creator1/9  "iz_pu_ref"
  [isb] -> Bus Creator1/6  "isb_pu"
  [isb_ref] -> Bus Creator1/5  "isb_pu_ref"
  [iz_ctrl_out] -> Bus Creator1/11  "iz_ctrl_out"
  [isc_ref] -> Bus Creator1/7  "isc_pu_ref"
  Bus Creator1/1 -> m_inner_current_tracking/1

== system afe_rst_ctrl/afe_abc_inv_psm_mod1/AFE_control/afe_control/data_to_worspace_module_1/pwr_meter ==
  Bus Creator1 : BusCreator  Inputs=4
  m_pwr_meter : Outport
  wires:
  [u_grid_pu_rms] -> Bus Creator1/2  "u_grid_pu_rms"
  Bus Creator1/1 -> m_pwr_meter/1
  [pwr_act_grid] -> Bus Creator1/3  "pwr_act_grid"
  [pwr_react_grid] -> Bus Creator1/4  "pwr_react_grid"
  [i_grid_pu_rms] -> Bus Creator1/1  "i_grid_pu_rms"

== system afe_rst_ctrl/afe_abc_inv_psm_mod1/AFE_control/afe_control/data_to_worspace_module_1/sequences_data ==
  Bus Creator1 : BusCreator  Inputs=11
  Demux : Demux  Outputs=3
  m_seq : Outport
  wires:
  Bus Creator1/1 -> m_seq/1
  Demux/3 -> Bus Creator1/3  "i_grid_neg_eta_ref"
  Demux/2 -> Bus Creator1/2  "i_grid_neg_xi_ref"
  Demux/1 -> Bus Creator1/1  "i_grid_pos_eta_ref"
  [v_grid_pos_xi_avg] -> Bus Creator1/4  "v_grid_pos_xi_avg"
  [v_grid_pos_eta_avg] -> Bus Creator1/5  "v_grid_pos_eta_avg"
  [v_grid_neg_xi_avg] -> Bus Creator1/6  "v_grid_neg_xi_avg"
  [v_grid_neg_eta_avg] -> Bus Creator1/7  "v_grid_neg_eta_avg"
  [i_grid_pos_xi_avg] -> Bus Creator1/8  "i_grid_pos_xi_avg"
  [i_grid_pos_eta_avg] -> Bus Creator1/9  "i_grid_pos_eta_avg"
  [i_grid_neg_xi_avg] -> Bus Creator1/10  "i_grid_neg_xi_avg"
  [i_grid_neg_eta_avg] -> Bus Creator1/11  "i_grid_neg_eta_avg"
  [i_grid_seq_ref] -> Demux/1

== system afe_rst_ctrl/afe_abc_inv_psm_mod1/AFE_control/afe_control/grid_voltage_phase_lock_loops/FHT-PLL_simulink ==
  ug_abc_pu : Inport
  pll_stageA : Subsystem
  pll_stageB : Subsystem
  gamma_grid_fht_pll : Outport
  omega_grid_fht_pll : Outport  Port=2
  wires:
  pll_stageB/1(gamma_grid_ddsrf_pll) -> pll_stageA/1(gamma_grid), gamma_grid_fht_pll/1
  pll_stageA/2(u_grid_eta) -> pll_stageB/2(u_grid_pos_eta)  "u_grid_pos_eta"
  pll_stageA/1(u_grid_xi) -> pll_stageB/1(u_grid_pos_xi)  "u_grid_pos_xi"
  pll_stageB/2(omega_grid_ddsrf_pll) -> omega_grid_fht_pll/1
  ug_abc_pu/1 -> pll_stageA/2(ug_abc_pu)

== system afe_rst_ctrl/afe_abc_inv_psm_mod1/AFE_control/afe_control/ig afe quantizzation and one step delay/ig afe quantizzation and one step delay ==
  ig_u_pu : Inport
  ig_v_pu : Inport  Port=2
  ig_w_pu : Inport  Port=3
  Gain4 : Gain  Gain=-1
  Gain5 : Gain  Gain=-1
  Gain6 : Gain  Gain=-1
  Quantizer1 : Quantizer  QuantizationInterval=param.meas.adc_quantization
  Quantizer2 : Quantizer  QuantizationInterval=param.meas.adc_quantization
  Quantizer4 : Quantizer  QuantizationInterval=param.meas.adc_quantization
  Unit Delay : UnitDelay  SampleTime=-1
  Unit Delay1 : UnitDelay  SampleTime=-1
  Unit Delay2 : UnitDelay  SampleTime=-1
  Zero-Order Hold : ZeroOrderHold  SampleTime=-1
  Zero-Order Hold1 : ZeroOrderHold  SampleTime=-1
  Zero-Order Hold2 : ZeroOrderHold  SampleTime=-1
  igd_u_pu : Outport
  igd_v_pu : Outport  Port=2
  igd_w_pu : Outport  Port=3
  wires:
  Quantizer1/1 -> Unit Delay1/1
  Quantizer4/1 -> Unit Delay/1
  Quantizer2/1 -> Unit Delay2/1
  ig_u_pu/1 -> Zero-Order Hold/1
  ig_v_pu/1 -> Zero-Order Hold1/1
  ig_w_pu/1 -> Zero-Order Hold2/1
  Unit Delay/1 -> Gain4/1
  Unit Delay1/1 -> Gain5/1
  Unit Delay2/1 -> Gain6/1
  Gain4/1 -> igd_u_pu/1
  Gain5/1 -> igd_v_pu/1
  Gain6/1 -> igd_w_pu/1
  Zero-Order Hold/1 -> Quantizer4/1
  Zero-Order Hold1/1 -> Quantizer1/1
  Zero-Order Hold2/1 -> Quantizer2/1

== system afe_rst_ctrl/afe_abc_inv_psm_mod1/AFE_control/afe_control/instantaneus_power/abc2alphabeta ==
  a : Inport
  b : Inport  Port=2
  c : Inport  Port=3
  Gain1 : Gain  Gain=-1/2
  Gain11 : Gain  Gain=-1/2
  Gain2 : Gain  Gain=0
  Gain3 : Gain  Gain=sqrt(3)/2
  Gain4 : Gain  Gain=-sqrt(3)/2
  Gain8 : Gain  Gain=2/3
  Gain9 : Gain  Gain=2/3
  Sum : Sum  Inputs=+++
  Sum1 : Sum  Inputs=+++
  "alpha " : Outport  VectorParamsAs1DForOutWhenUnconnected=off
  "beta " : Outport  Port=2  VectorParamsAs1DForOutWhenUnconnected=off
  wires:
  Gain3/1 -> Sum1/2
  Gain2/1 -> Sum1/1
  Gain11/1 -> Sum/2
  Gain4/1 -> Sum1/3
  Sum1/1 -> Gain9/1
  Gain8/1 -> "alpha "/1
  Sum/1 -> Gain8/1
  c/1 -> Gain4/1, Gain1/1
  Gain9/1 -> "beta "/1
  b/1 -> Gain3/1, Gain11/1
  Gain1/1 -> Sum/3
  a/1 -> Gain2/1, Sum/1

== system afe_rst_ctrl/afe_abc_inv_psm_mod1/AFE_control/afe_control/instantaneus_power/abc2alphabeta  ==
  a : Inport
  b : Inport  Port=2
  c : Inport  Port=3
  Gain1 : Gain  Gain=-1/2
  Gain11 : Gain  Gain=-1/2
  Gain2 : Gain  Gain=0
  Gain3 : Gain  Gain=sqrt(3)/2
  Gain4 : Gain  Gain=-sqrt(3)/2
  Gain8 : Gain  Gain=2/3
  Gain9 : Gain  Gain=2/3
  Sum : Sum  Inputs=+++
  Sum1 : Sum  Inputs=+++
  "alpha " : Outport  VectorParamsAs1DForOutWhenUnconnected=off
  "beta " : Outport  Port=2  VectorParamsAs1DForOutWhenUnconnected=off
  wires:
  a/1 -> Sum/1, Gain2/1
  Gain2/1 -> Sum1/1
  Gain9/1 -> "beta "/1
  Gain11/1 -> Sum/2
  c/1 -> Gain1/1, Gain4/1
  Sum/1 -> Gain8/1
  Sum1/1 -> Gain9/1
  Gain1/1 -> Sum/3
  Gain3/1 -> Sum1/2
  Gain4/1 -> Sum1/3
  Gain8/1 -> "alpha "/1
  b/1 -> Gain11/1, Gain3/1

== system afe_rst_ctrl/afe_abc_inv_psm_mod1/AFE_control/afe_control/instantaneus_power/moving_avarage_p ==
  in : Inport
  Gain : Gain  Gain=param.afe.ctrl.rms.n1-1
  Gain1 : Gain  Gain=1/param.afe.ctrl.rms.n1
  Sum : Sum  Inputs=|++
  Unit Delay : UnitDelay  SampleTime=-1
  out : Outport  VectorParamsAs1DForOutWhenUnconnected=off
  wires:
  Gain/1 -> Sum/2
  Gain1/1 -> out/1, Unit Delay/1
  in/1 -> Sum/1
  Unit Delay/1 -> Gain/1
  Sum/1 -> Gain1/1

== system afe_rst_ctrl/afe_abc_inv_psm_mod1/AFE_control/afe_control/instantaneus_power/moving_avarage_q ==
  in : Inport
  Gain : Gain  Gain=param.afe.ctrl.rms.n1-1
  Gain1 : Gain  Gain=1/param.afe.ctrl.rms.n1
  Sum : Sum  Inputs=|++
  Unit Delay : UnitDelay  SampleTime=-1
  out : Outport  VectorParamsAs1DForOutWhenUnconnected=off
  wires:
  Sum/1 -> Gain1/1
  Unit Delay/1 -> Gain/1
  in/1 -> Sum/1
  Gain1/1 -> Unit Delay/1, out/1
  Gain/1 -> Sum/2

== system afe_rst_ctrl/afe_abc_inv_psm_mod1/AFE_control/afe_control/instantaneus_power/rms ==
  In1 : Inport
  Gain : Gain  Gain=param.afe.ctrl.rms.n10-1
  Gain1 : Gain  Gain=1/param.afe.ctrl.rms.n10
  Math Function : Math  Operator=magnitude^2  SignedPower=on
  Sqrt : Sqrt
  Sum : Sum  Inputs=|++
  Unit Delay : UnitDelay  SampleTime=-1
  Out1 : Outport  VectorParamsAs1DForOutWhenUnconnected=off
  wires:
  In1/1 -> Math Function/1
  Sum/1 -> Gain1/1
  Gain1/1 -> Sqrt/1, Unit Delay/1
  Unit Delay/1 -> Gain/1
  Math Function/1 -> Sum/1
  Sqrt/1 -> Out1/1
  Gain/1 -> Sum/2

== system afe_rst_ctrl/afe_abc_inv_psm_mod1/AFE_control/afe_control/instantaneus_power/rms1 ==
  In1 : Inport
  Gain : Gain  Gain=param.afe.ctrl.rms.n10-1
  Gain1 : Gain  Gain=1/param.afe.ctrl.rms.n10
  Math Function : Math  Operator=magnitude^2  SignedPower=on
  Sqrt : Sqrt
  Sum : Sum  Inputs=|++
  Unit Delay : UnitDelay  SampleTime=-1
  Out1 : Outport  VectorParamsAs1DForOutWhenUnconnected=off
  wires:
  Gain/1 -> Sum/2
  Sqrt/1 -> Out1/1
  Math Function/1 -> Sum/1
  Unit Delay/1 -> Gain/1
  Gain1/1 -> Unit Delay/1, Sqrt/1
  Sum/1 -> Gain1/1
  In1/1 -> Math Function/1

== system afe_rst_ctrl/afe_abc_inv_psm_mod1/AFE_control/afe_control/instantaneus_power/rms2 ==
  In1 : Inport
  Gain : Gain  Gain=param.afe.ctrl.rms.n10-1
  Gain1 : Gain  Gain=1/param.afe.ctrl.rms.n10
  Math Function : Math  Operator=magnitude^2  SignedPower=on
  Sqrt : Sqrt
  Sum : Sum  Inputs=|++
  Unit Delay : UnitDelay  SampleTime=-1
  Out1 : Outport  VectorParamsAs1DForOutWhenUnconnected=off
  wires:
  In1/1 -> Math Function/1
  Sum/1 -> Gain1/1
  Gain1/1 -> Sqrt/1, Unit Delay/1
  Unit Delay/1 -> Gain/1
  Math Function/1 -> Sum/1
  Sqrt/1 -> Out1/1
  Gain/1 -> Sum/2

== system afe_rst_ctrl/afe_abc_inv_psm_mod1/AFE_control/afe_control/instantaneus_power/rms3 ==
  In1 : Inport
  Gain : Gain  Gain=param.afe.ctrl.rms.n10-1
  Gain1 : Gain  Gain=1/param.afe.ctrl.rms.n10
  Math Function : Math  Operator=magnitude^2  SignedPower=on
  Sqrt : Sqrt
  Sum : Sum  Inputs=|++
  Unit Delay : UnitDelay  SampleTime=-1
  Out1 : Outport  VectorParamsAs1DForOutWhenUnconnected=off
  wires:
  Gain/1 -> Sum/2
  Sqrt/1 -> Out1/1
  Math Function/1 -> Sum/1
  Unit Delay/1 -> Gain/1
  Gain1/1 -> Unit Delay/1, Sqrt/1
  Sum/1 -> Gain1/1
  In1/1 -> Math Function/1

== system afe_rst_ctrl/afe_abc_inv_psm_mod1/AFE_control/afe_control/instantaneus_power/rms4 ==
  In1 : Inport
  Gain : Gain  Gain=param.afe.ctrl.rms.n10-1
  Gain1 : Gain  Gain=1/param.afe.ctrl.rms.n10
  Math Function : Math  Operator=magnitude^2  SignedPower=on
  Sqrt : Sqrt
  Sum : Sum  Inputs=|++
  Unit Delay : UnitDelay  SampleTime=-1
  Out1 : Outport  VectorParamsAs1DForOutWhenUnconnected=off
  wires:
  In1/1 -> Math Function/1
  Sum/1 -> Gain1/1
  Gain1/1 -> Sqrt/1, Unit Delay/1
  Unit Delay/1 -> Gain/1
  Math Function/1 -> Sum/1
  Sqrt/1 -> Out1/1
  Gain/1 -> Sum/2

== system afe_rst_ctrl/afe_abc_inv_psm_mod1/AFE_control/afe_control/instantaneus_power/rms5 ==
  In1 : Inport
  Gain : Gain  Gain=param.afe.ctrl.rms.n10-1
  Gain1 : Gain  Gain=1/param.afe.ctrl.rms.n10
  Math Function : Math  Operator=magnitude^2  SignedPower=on
  Sqrt : Sqrt
  Sum : Sum  Inputs=|++
  Unit Delay : UnitDelay  SampleTime=-1
  Out1 : Outport  VectorParamsAs1DForOutWhenUnconnected=off
  wires:
  Gain/1 -> Sum/2
  Sqrt/1 -> Out1/1
  Math Function/1 -> Sum/1
  Unit Delay/1 -> Gain/1
  Gain1/1 -> Unit Delay/1, Sqrt/1
  Sum/1 -> Gain1/1
  In1/1 -> Math Function/1

== system afe_rst_ctrl/afe_abc_inv_psm_mod1/AFE_control/afe_control/is afe quantizzation and one step delay/is afe quantizzation and one step delay ==
  is_u_pu : Inport
  is_v_pu : Inport  Port=2
  is_w_pu : Inport  Port=3
  Quantizer : Quantizer  QuantizationInterval=param.meas.adc_quantization
  Quantizer1 : Quantizer  QuantizationInterval=param.meas.adc_quantization
  Quantizer2 : Quantizer  QuantizationInterval=param.meas.adc_quantization
  Unit Delay : UnitDelay  SampleTime=-1
  Unit Delay1 : UnitDelay  SampleTime=-1
  Unit Delay2 : UnitDelay  SampleTime=-1
  Zero-Order Hold : ZeroOrderHold  SampleTime=-1
  Zero-Order Hold1 : ZeroOrderHold  SampleTime=-1
  Zero-Order Hold2 : ZeroOrderHold  SampleTime=-1
  isd_u_pu : Outport
  isd_v_pu : Outport  Port=2
  isd_w_pu : Outport  Port=3
  wires:
  Unit Delay/1 -> isd_u_pu/1
  Unit Delay1/1 -> isd_v_pu/1
  Unit Delay2/1 -> isd_w_pu/1
  Quantizer/1 -> Unit Delay/1
  Quantizer1/1 -> Unit Delay1/1
  Quantizer2/1 -> Unit Delay2/1
  is_u_pu/1 -> Zero-Order Hold/1
  is_v_pu/1 -> Zero-Order Hold1/1
  is_w_pu/1 -> Zero-Order Hold2/1
  Zero-Order Hold/1 -> Quantizer/1
  Zero-Order Hold1/1 -> Quantizer1/1
  Zero-Order Hold2/1 -> Quantizer2/1

== system afe_rst_ctrl/afe_abc_inv_psm_mod1/AFE_control/afe_control/phase_compensation_1/alignment_eval_afe1 ==
  local_time : Inport
  master_time : Inport  Port=2
  Constant : Constant  Value=0
  Gain : Gain  Gain=-1
  Sum : Sum  Inputs=|+-
  pi : Subsystem  mask{kp=param.ctrl.kp_align, ki=param.ctrl.ki_align*param.glb_time.ts_afe, lim_up=param.ctrl.lim_up_align, lim_down=param.ctrl.lim_down_align}
      mask prompts: ki "ki*ts"
      mask Display:
      | disp('pi()');
      | port_label('input', 1, 'u_ref');
      | port_label('input', 2, 'u');
      | port_label('output', 1, 'y');
  dp : Outport
  wires:
  master_time/1 -> Sum/1
  Sum/1 -> Gain/1
  Constant/1 -> pi/1(u_ref)
  local_time/1 -> Sum/2
  Gain/1 -> pi/2(u)
  pi/1(y) -> dp/1

== system afe_rst_ctrl/afe_abc_inv_psm_mod1/AFE_control/afe_control/ug afe quantizzation and one step delay/ug afe quantizzation and one step delay ==
  ug_u_pu : Inport
  ug_v_pu : Inport  Port=2
  ug_w_pu : Inport  Port=3
  Quantizer1 : Quantizer  QuantizationInterval=param.meas.adc_quantization
  Quantizer2 : Quantizer  QuantizationInterval=param.meas.adc_quantization
  Quantizer4 : Quantizer  QuantizationInterval=param.meas.adc_quantization
  Unit Delay : UnitDelay  SampleTime=-1
  Unit Delay1 : UnitDelay  SampleTime=-1
  Unit Delay2 : UnitDelay  SampleTime=-1
  Zero-Order Hold : ZeroOrderHold  SampleTime=-1
  Zero-Order Hold1 : ZeroOrderHold  SampleTime=-1
  Zero-Order Hold2 : ZeroOrderHold  SampleTime=-1
  ugd_u_pu : Outport
  ugd_v_pu : Outport  Port=2
  ugd_w_pu : Outport  Port=3
  wires:
  Unit Delay/1 -> ugd_u_pu/1
  Unit Delay1/1 -> ugd_v_pu/1
  Unit Delay2/1 -> ugd_w_pu/1
  Quantizer4/1 -> Unit Delay/1
  Quantizer1/1 -> Unit Delay1/1
  Quantizer2/1 -> Unit Delay2/1
  ug_w_pu/1 -> Zero-Order Hold2/1
  ug_v_pu/1 -> Zero-Order Hold1/1
  ug_u_pu/1 -> Zero-Order Hold/1
  Zero-Order Hold/1 -> Quantizer4/1
  Zero-Order Hold1/1 -> Quantizer1/1
  Zero-Order Hold2/1 -> Quantizer2/1
